simulink model "corrected_circuit"  (R2025a)
settings: Solver=ode23t  StartTime=0.0  StopTime=8.1  MaxStep=0.001  RelTol=1e-7  AbsTol=1e-9
libraries: fl_lib x38, nesl_utility x8
settings Model: Creator=lelala271  LastModifiedBy=lelala271
settings DataIOCC: SaveOutput=off  SignalLogging=off  OutputOption=SpecifiedOutputTimes  OutputTimes=0:0.0005:8.1

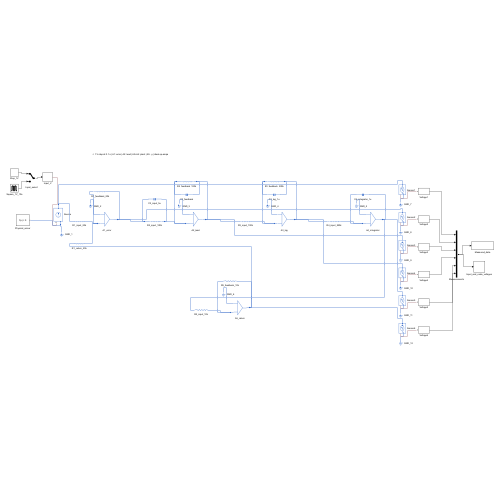
[thumbnail: Simulink's stored preview of the top-level diagram]
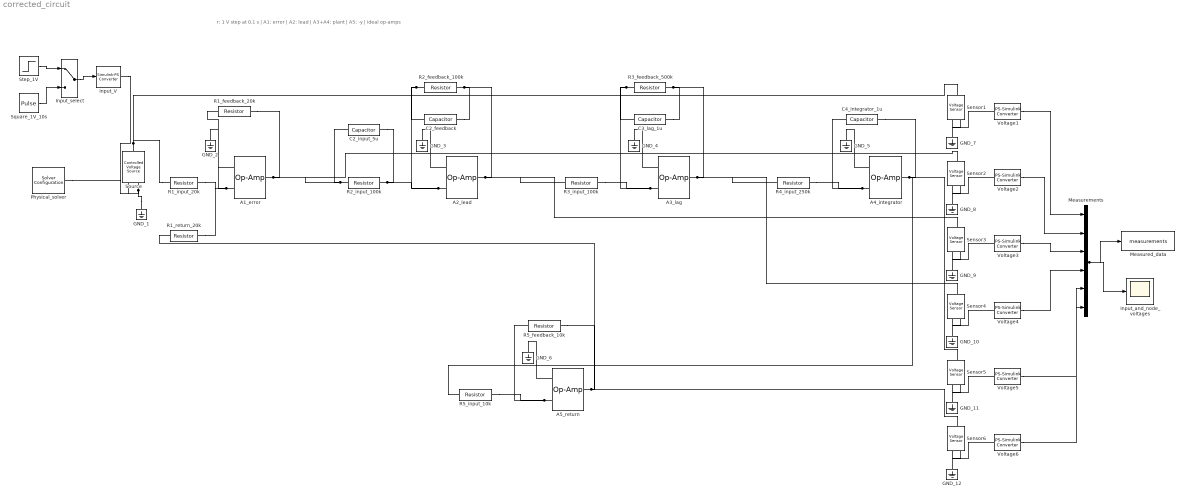
== system corrected_circuit ==
  note: r: 1 V step at 0.1 s | A1: error | A2: lead | A3+A4: plant | A5: -y | ideal op-amps
  A1_error : fl_lib/Electrical/Electrical Elements/Op-Amp  outI_specify=off  outI_priority=None  outI=0 A  outI_nominal_specify=off  outI_nominal_value=1  outI_nominal_unit=A
  A2_lead : fl_lib/Electrical/Electrical Elements/Op-Amp  outI_specify=off  outI_priority=None  outI=0 A  outI_nominal_specify=off  outI_nominal_value=1  outI_nominal_unit=A
  A3_lag : fl_lib/Electrical/Electrical Elements/Op-Amp  outI_specify=off  outI_priority=None  outI=0 A  outI_nominal_specify=off  outI_nominal_value=1  outI_nominal_unit=A
  A4_integrator : fl_lib/Electrical/Electrical Elements/Op-Amp  outI_specify=off  outI_priority=None  outI=0 A  outI_nominal_specify=off  outI_nominal_value=1  outI_nominal_unit=A
  A5_return : fl_lib/Electrical/Electrical Elements/Op-Amp  outI_specify=off  outI_priority=None  outI=0 A  outI_nominal_specify=off  outI_nominal_value=1  outI_nominal_unit=A
  C2_feedback : fl_lib/Electrical/Electrical Elements/Capacitor  c=2.5e-7 F  r=0 Ohm  g=0 1/Ohm  i_specify=off  i_priority=None  i=0 A  i_nominal_specify=off  i_nominal_value=1  i_nominal_unit=A  v_specify=off  v_priority=None  v=0 V  v_nominal_specify=off  v_nominal_value=1  v_nominal_unit=V  vc_specify=off  vc_priority=High  vc=0 V  vc_nominal_specify=off  vc_nominal_value=1  vc_nominal_unit=V
  C2_input_5u : fl_lib/Electrical/Electrical Elements/Capacitor  c=5e-06 F  r=0 Ohm  g=0 1/Ohm  i_specify=off  i_priority=None  i=0 A  i_nominal_specify=off  i_nominal_value=1  i_nominal_unit=A  v_specify=off  v_priority=None  v=0 V  v_nominal_specify=off  v_nominal_value=1  v_nominal_unit=V  vc_specify=off  vc_priority=High  vc=0 V  vc_nominal_specify=off  vc_nominal_value=1  vc_nominal_unit=V
  C3_lag_1u : fl_lib/Electrical/Electrical Elements/Capacitor  c=1e-06 F  r=0 Ohm  g=0 1/Ohm  i_specify=off  i_priority=None  i=0 A  i_nominal_specify=off  i_nominal_value=1  i_nominal_unit=A  v_specify=off  v_priority=None  v=0 V  v_nominal_specify=off  v_nominal_value=1  v_nominal_unit=V  vc_specify=off  vc_priority=High  vc=0 V  vc_nominal_specify=off  vc_nominal_value=1  vc_nominal_unit=V
  C4_integrator_1u : fl_lib/Electrical/Electrical Elements/Capacitor  c=1e-06 F  r=0 Ohm  g=0 1/Ohm  i_specify=off  i_priority=None  i=0 A  i_nominal_specify=off  i_nominal_value=1  i_nominal_unit=A  v_specify=off  v_priority=None  v=0 V  v_nominal_specify=off  v_nominal_value=1  v_nominal_unit=V  vc_specify=off  vc_priority=High  vc=0 V  vc_nominal_specify=off  vc_nominal_value=1  vc_nominal_unit=V
  GND_{1..12} (12 alike) : fl_lib/Electrical/Electrical Elements/Electrical Reference
  Input_V : nesl_utility/Simulink-PS Converter  PhysicalDomain=network_engine_domain  SubClassName=ps_input  LeftPortType=input  RightPortType=output  PseudoPeriodic=off  Frequencies=[]  NoiseDistribution=none  NoiseParameters=[]  Unit=V  AffineConversion=off  FilteringAndDerivatives=filter  SimscapeFilterOrder=1  InputFilterTimeConstant=1e-4  UdotUserProvided=0
  Input_and_node_voltages : Scope
  Input_select : ManualSwitch
  Measured_data : ToWorkspace  VariableName=measurements  SaveFormat=Timeseries  SampleTime=-1
  Measurements : Mux  Inputs=6
  Physical_solver : nesl_utility/Solver Configuration  PhysicalDomain=network_engine_domain  SubClassName=solver  LeftPortType=input  RightPortType=generic  Tones=[]  Harmonics=[]  SimulateNoise=off  Profile=off  UseLocalSampling=off  EnableSwitchedLinearOptims=on  FrequencyDomain=off  UseCCode=off  RelTol=0.001  AbsTol=0.001  MinStep=1e-09  ToWorkspace=off  RevertToSquareIcSolve=off  NumHomotopyIterations=100  PhasorMode=off  PhasorModeNumHarmonics=1  ConsistencySolver=NEWTON_XTOL_AFTER_FTOL  IndexReductionMethod=DerivativeReplacement  DoDC=off  ResidualTolerance=1e-09  ConsistencyTolSource=GLOBAL  ConsistencyAbsTol=0.001  ConsistencyRelTol=0.001  ConsistencyTolFactor=0.001  UseLocalSolver=off  LocalSolverChoice=NE_BACKWARD_EULER_ADVANCER  ResolveIndetEquations=on  FunctionEvalNumThread=1  LocalSolverSampleTime=0.001  DoFixedCost=off  MaxNonlinIter=3  MaxModeIter=2  ComputeImpulses=off  ImpulseIterations=2  LinearAlgebra=auto  LinearAlgebraNumThread=0  EquationFormulation=NE_TIME_EF  DelaysMemoryBudget=1024  AutomaticFiltering=on  FilteringTimeConstant=0.001  PartitionStorageMethod=AS_NEEDED  PartitionMemoryBudget=1024  PartitionMethod=ROBUST  MultibodyUseLocalSolver=off  MultibodyLocalSolverChoice=ODE1  MultibodyLocalSolverSampleTime=0.001
  R1_feedback_20k : fl_lib/Electrical/Electrical Elements/Resistor  R=20000 Ohm  i_specify=off  i_priority=None  i=0 A  i_nominal_specify=off  i_nominal_value=1  i_nominal_unit=A  v_specify=off  v_priority=None  v=0 V  v_nominal_specify=off  v_nominal_value=1  v_nominal_unit=V
  R1_input_20k : fl_lib/Electrical/Electrical Elements/Resistor  R=20000 Ohm  i_specify=off  i_priority=None  i=0 A  i_nominal_specify=off  i_nominal_value=1  i_nominal_unit=A  v_specify=off  v_priority=None  v=0 V  v_nominal_specify=off  v_nominal_value=1  v_nominal_unit=V
  R1_return_20k : fl_lib/Electrical/Electrical Elements/Resistor  R=20000 Ohm  i_specify=off  i_priority=None  i=0 A  i_nominal_specify=off  i_nominal_value=1  i_nominal_unit=A  v_specify=off  v_priority=None  v=0 V  v_nominal_specify=off  v_nominal_value=1  v_nominal_unit=V
  R2_feedback_100k : fl_lib/Electrical/Electrical Elements/Resistor  R=100000 Ohm  i_specify=off  i_priority=None  i=0 A  i_nominal_specify=off  i_nominal_value=1  i_nominal_unit=A  v_specify=off  v_priority=None  v=0 V  v_nominal_specify=off  v_nominal_value=1  v_nominal_unit=V
  R2_input_100k : fl_lib/Electrical/Electrical Elements/Resistor  R=100000 Ohm  i_specify=off  i_priority=None  i=0 A  i_nominal_specify=off  i_nominal_value=1  i_nominal_unit=A  v_specify=off  v_priority=None  v=0 V  v_nominal_specify=off  v_nominal_value=1  v_nominal_unit=V
  R3_feedback_500k : fl_lib/Electrical/Electrical Elements/Resistor  R=500000 Ohm  i_specify=off  i_priority=None  i=0 A  i_nominal_specify=off  i_nominal_value=1  i_nominal_unit=A  v_specify=off  v_priority=None  v=0 V  v_nominal_specify=off  v_nominal_value=1  v_nominal_unit=V
  R3_input_100k : fl_lib/Electrical/Electrical Elements/Resistor  R=100000 Ohm  i_specify=off  i_priority=None  i=0 A  i_nominal_specify=off  i_nominal_value=1  i_nominal_unit=A  v_specify=off  v_priority=None  v=0 V  v_nominal_specify=off  v_nominal_value=1  v_nominal_unit=V
  R4_input_250k : fl_lib/Electrical/Electrical Elements/Resistor  R=250000 Ohm  i_specify=off  i_priority=None  i=0 A  i_nominal_specify=off  i_nominal_value=1  i_nominal_unit=A  v_specify=off  v_priority=None  v=0 V  v_nominal_specify=off  v_nominal_value=1  v_nominal_unit=V
  R5_feedback_10k : fl_lib/Electrical/Electrical Elements/Resistor  R=10000 Ohm  i_specify=off  i_priority=None  i=0 A  i_nominal_specify=off  i_nominal_value=1  i_nominal_unit=A  v_specify=off  v_priority=None  v=0 V  v_nominal_specify=off  v_nominal_value=1  v_nominal_unit=V
  R5_input_10k : fl_lib/Electrical/Electrical Elements/Resistor  R=10000 Ohm  i_specify=off  i_priority=None  i=0 A  i_nominal_specify=off  i_nominal_value=1  i_nominal_unit=A  v_specify=off  v_priority=None  v=0 V  v_nominal_specify=off  v_nominal_value=1  v_nominal_unit=V
  Sensor{1..6} (6 alike) : fl_lib/Electrical/Electrical Sensors/Voltage Sensor
  Source : fl_lib/Electrical/Electrical Sources/Controlled Voltage Source
  Square_1V_10s : DiscretePulseGenerator  PulseType=Time based  Period=10  PulseWidth=50  PhaseDelay=0.1
  Step_1V : Step  Time=0.1  SampleTime=0
  Voltage{1..6} (6 alike) : nesl_utility/PS-Simulink Converter  PhysicalDomain=network_engine_domain  SubClassName=ps_output  LeftPortType=input  RightPortType=output  PseudoPeriodic=off  Frequencies=[]  VectorFormat=inherit  Unit=V  AffineConversion=off
  wires:
  Step_1V/1 -> Input_select/1
  Square_1V_10s/1 -> Input_select/2
  Input_select/1 -> Input_V/1
  Voltage1/1 -> Measurements/1
  Voltage2/1 -> Measurements/2
  Voltage3/1 -> Measurements/3
  Voltage4/1 -> Measurements/4
  Voltage5/1 -> Measurements/5
  Voltage6/1 -> Measurements/6
  Measurements/1 -> Measured_data/1, Input_and_node_voltages/1
  connections:
  Input_V/RConn1 -- Source/RConn1
  GND_1/LConn1 -- Source/RConn2 -- Physical_solver/RConn1
  A1_error/LConn1 -- GND_2/LConn1
  R1_input_20k/LConn1 -- Source/LConn1 -- Sensor1/LConn1
  R1_input_20k/RConn1 -- R1_feedback_20k/LConn1 -- A1_error/LConn2 -- R1_return_20k/RConn1
  R1_feedback_20k/RConn1 -- R2_input_100k/LConn1 -- C2_input_5u/LConn1 -- A1_error/RConn1 -- Sensor2/LConn1
  A2_lead/LConn1 -- GND_3/LConn1
  A2_lead/LConn2 -- R2_input_100k/RConn1 -- C2_input_5u/RConn1 -- R2_feedback_100k/LConn1 -- C2_feedback/LConn1
  R2_feedback_100k/RConn1 -- C2_feedback/RConn1 -- R3_input_100k/LConn1 -- A2_lead/RConn1 -- Sensor3/LConn1
  A3_lag/LConn1 -- GND_4/LConn1
  A3_lag/LConn2 -- R3_input_100k/RConn1 -- R3_feedback_500k/LConn1 -- C3_lag_1u/LConn1
  R3_feedback_500k/RConn1 -- C3_lag_1u/RConn1 -- R4_input_250k/LConn1 -- A3_lag/RConn1 -- Sensor4/LConn1
  A4_integrator/LConn1 -- GND_5/LConn1
  A4_integrator/LConn2 -- R4_input_250k/RConn1 -- C4_integrator_1u/LConn1
  C4_integrator_1u/RConn1 -- R5_input_10k/LConn1 -- A4_integrator/RConn1 -- Sensor5/LConn1
  A5_return/LConn1 -- GND_6/LConn1
  A5_return/LConn2 -- R5_input_10k/RConn1 -- R5_feedback_10k/LConn1
  R5_feedback_10k/RConn1 -- R1_return_20k/LConn1 -- A5_return/RConn1 -- Sensor6/LConn1
  Sensor1/RConn2 -- GND_7/LConn1
  Sensor1/RConn1 -- Voltage1/LConn1
  Sensor2/RConn2 -- GND_8/LConn1
  Sensor2/RConn1 -- Voltage2/LConn1
  Sensor3/RConn2 -- GND_9/LConn1
  Sensor3/RConn1 -- Voltage3/LConn1
  Sensor4/RConn2 -- GND_10/LConn1
  Sensor4/RConn1 -- Voltage4/LConn1
  Sensor5/RConn2 -- GND_11/LConn1
  Sensor5/RConn1 -- Voltage5/LConn1
  Sensor6/RConn2 -- GND_12/LConn1
  Sensor6/RConn1 -- Voltage6/LConn1
